simulink model "homeMobileManipulator"  (R2026a)
settings: Solver=ode4  StartTime=0  StopTime=Inf  FixedStep=cfg.rates.plant  MaxStep=cfg.rates.plant  AbsTol=1e-8
PostLoadFcn:
  | hmmSetup;
InitFcn:
  | hmmInitializeRun(bdroot);
values from neighbouring files (symbols this model uses):
  armJointLimits = zeros(numel(idx.arm), 2)    [hmmSetup.m]
  cfg = app.RunCfg    [HomeMobileManipulatorApp.m]    (also in HomeMobileManipulatorExample.m = params.cfg; hmmSetup.m = hmmConfig(); setupParams.m = data.cfg)
undefined symbols (not defined in the file or in its folder): actionQueueInit, actorNameTable, Angle, apertureMap, armPlanInit, Axis, basePlanInit, Custom, Extent, gray, gripperCoupling, invalidRayHits, movableRegistry, objectTargetInit, perceptionStatusInit, placeTargetInit, Position, robotStateInit, Sim3dSensor
libraries: robotmaniplib x20, robotcorelib x18, simulink x9, sim3dcameralib x6, sim3dgroundtruthsensorlib x4, dspmtrx3 x3, slpidlib x3, sim3dlib x3, hdlsllib x2, robotsim3dlib x1
(part 3 of 6)

== system homeMobileManipulator/MobileManipulator/Plant/RobotActor ==
  note: Scene frame -> render frame. The Simulation 3D Robot block negates y on EVERY LINK of
      | the tree it is given, while every Simulation 3D Actor and Camera here takes its
      | Translation as given - so the conversion is one frame change too many. RobotTree is
      | therefore handed renderRobot, a y-mirrored COPY of the tree (hmmMirrorTree), and driven
      | with the TRUE configuration: FK of the mirrored tree is M*FK(q)*M for every q, so the
      | block's own negation cancels exactly. This replaces a Gain that pre-negated the base y
      | and yaw only, which fixed 3 of 15 degrees of freedom and left the arm rendering as its
      | own mirror image. RENDER PATH ONLY - renderRobot's joint angles do not mean what they
      | say and its frames are left-handed; control, planning, perception and every FK
      | measurement use data.robot.
  GripperJointVector : Inport
  ArmJointPos : Inport  Port=2
  BasePose : Inport  Port=3
  TargetActorId : Inport  Port=4
  ActivateGrasp : Inport  Port=5
  TargetActorName : Inport  Port=6
  ActorRotationCol : Reshape  OutputDimensionality=Customize  OutputDimensions=[3 1]
  ActorTranslationCol : Reshape  OutputDimensionality=Customize  OutputDimensions=[3 1]
  AttachedActorSelect : Switch  Criteria=u2 ~= 0
  ConfigMux : Mux  Inputs=3
  ConfigRow : Reshape  OutputDimensionality=Customize  OutputDimensions=[1 15]
  NoActor : Constant  Value=cfg.actor.noneId  OutDataTypeStr=uint8
  ReleaseSettle : MATLAB Function  TreatAsAtomicUnit=on  SystemSampleTime=cfg.rates.scene
  RobotTree : robotsim3dlib/Simulation 3D Robot  actorInputType=RigidBodyTree Object  RigidBodyTree=renderRobot  ActorName=SimulinkVehicle1  existActorChekBox=off  initialTrans=[0 0 0]  initialRot=[0 0 0]  initialConfig=[cfg.base.initialPose(:)', cfg.arm.stowConfig, zeros(1,6)]  EndEffector=tcp_frame  eeOffsetInpChekBox=off  eeTargetTrans=carryTranslation  eeTargetRot=[0 0 0]  enableRegionGraspChekBox=off  regionGraspInpChekBox=off  eeTargTransDiff=[0.2 0.2 0.2]  eeTargRotDiff=[0 0 0]  enableVisualVisualization=on  enableCollisionVisualization=off  collisionGeomColor=[0 1 0]  collisionGeomTransp=0.1  inpConfEnbVal=on  inpGraspEnbVal=on  inpTransEnbVal=off  outConfEnbVal=off  outGraspEnbVal=on  outTransEnbVal=on  SampleTime=cfg.rates.scene  ActorType=SimulinkVehicle  ID=1  aMode=6  ActorTag=SimulinkVehicle1  Mesh=RigidBodyTree
      link override MATLAB System: RobotActorName=ActorName  EndEffectorName=EndEffector
  SettleDzOpen : Terminator
  RobotConfig : Outport
  ActorTranslation : Outport  Port=2
  ActorRotation : Outport  Port=3
  IsGrasped : Outport  Port=4
  AttachedActorId : Outport  Port=5
  wires:
  ActorRotationCol/1 -> ActorRotation/1  "ActorRotation"
  ActorTranslationCol/1 -> ActorTranslation/1  "ActorTranslation"
  AttachedActorSelect/1 -> AttachedActorId/1  "AttachedActorId"
  RobotTree/3 -> ActorRotationCol/1  "ActorRotationRow"
  RobotTree/2 -> ActorTranslationCol/1  "ActorTranslationRow"
  RobotTree/1 -> ReleaseSettle/1(IsGrasped), AttachedActorSelect/2, IsGrasped/1  "IsGrasped"
  TargetActorId/1 -> AttachedActorSelect/1, ReleaseSettle/2(TargetActorId)
  NoActor/1 -> AttachedActorSelect/3
  TargetActorName/1 -> RobotTree/2  "TargetActorName"
  ConfigRow/1 -> RobotTree/1, ReleaseSettle/3(RobotConfig), RobotConfig/1  "RobotConfig"
  ConfigMux/1 -> ConfigRow/1
  ActivateGrasp/1 -> RobotTree/3
  GripperJointVector/1 -> ConfigMux/3
  ArmJointPos/1 -> ConfigMux/2
  BasePose/1 -> ConfigMux/1
  ReleaseSettle/1(SettleDz) -> SettleDzOpen/1

== system homeMobileManipulator/MobileManipulator/Plant/StateReport ==
  BasePose : Inport
  BaseTwist : Inport  Port=2
  WheelSpeeds : Inport  Port=3
  ArmJointPos : Inport  Port=4
  ArmJointVel : Inport  Port=5
  GripperAperture : Inport  Port=6
  GripperDriverAngle : Inport  Port=7
  ToolTranslation : Inport  Port=8
  ToolRotation : Inport  Port=9
  ActorTranslation : Inport  Port=10
  ActorRotation : Inport  Port=11
  AttachedActorId : Inport  Port=12
  IsGrasped : Inport  Port=13
  ReportTime : DigitalClock  SampleTime=cfg.rates.plant
  RobotStateBus : BusCreator  Inputs=15  OutDataTypeStr=Bus: RobotState
      settings: InheritFromInputs=off
  StateValid : Constant  OutDataTypeStr=boolean
  RobotState : Outport
  wires:
  StateValid/1 -> RobotStateBus/15
  ReportTime/1 -> RobotStateBus/14
  IsGrasped/1 -> RobotStateBus/13
  AttachedActorId/1 -> RobotStateBus/12
  ActorRotation/1 -> RobotStateBus/11
  ActorTranslation/1 -> RobotStateBus/10
  ToolRotation/1 -> RobotStateBus/9
  ToolTranslation/1 -> RobotStateBus/8
  ArmJointVel/1 -> RobotStateBus/5
  ArmJointPos/1 -> RobotStateBus/4
  WheelSpeeds/1 -> RobotStateBus/3
  GripperDriverAngle/1 -> RobotStateBus/7
  BaseTwist/1 -> RobotStateBus/2
  GripperAperture/1 -> RobotStateBus/6
  BasePose/1 -> RobotStateBus/1
  RobotStateBus/1 -> RobotState/1

== system homeMobileManipulator/MobileManipulator/Plant/ToolKinematics ==
  RobotConfig : Inport
  GraspFramePose : robotmaniplib/Get Transform  RigidBodyTree=robot  SourceBody=grasp_frame  TargetBody=map  SimulateUsing=Code generation
  GraspRotationUnused : Terminator
  GraspToEuler : robotcorelib/Coordinate Transformation Conversion  InputRepresentation=Homogeneous Transformation  InputEulerSequence=ZYX  ShowTrVecInputPort=on  OutputRepresentation=Euler Angles  OutputEulerSequence=XYZ  ShowTrVecOutputPort=on  SimulateUsing=Code generation
  TcpPose : robotmaniplib/Get Transform  RigidBodyTree=robot  SourceBody=tcp_frame  TargetBody=map  SimulateUsing=Code generation
  TcpToEuler : robotcorelib/Coordinate Transformation Conversion  InputRepresentation=Homogeneous Transformation  InputEulerSequence=ZYX  ShowTrVecInputPort=on  OutputRepresentation=Euler Angles  OutputEulerSequence=XYZ  ShowTrVecOutputPort=on  SimulateUsing=Code generation
  ToolTranslation : Outport
  ToolRotation : Outport  Port=2
  GraspFramePos : Outport  Port=3
  wires:
  GraspToEuler/1 -> GraspRotationUnused/1
  TcpToEuler/1 -> ToolRotation/1  "ToolRotation"
  GraspFramePose/1 -> GraspToEuler/1  "GraspTransform"
  TcpPose/1 -> TcpToEuler/1  "TcpTransform"
  TcpToEuler/2 -> ToolTranslation/1  "ToolTranslation"
  RobotConfig/1 -> TcpPose/1, GraspFramePose/1
  GraspToEuler/2 -> GraspFramePos/1  "GraspFramePos"

== system homeMobileManipulator/MobileManipulator/SafetyMonitor/BaseLimitChecks ==
  BaseTwist : Inport
  AbsAccel : Abs
  AbsTwist : Abs
  AccelExceeded : RelationalOperator  Operator=>
  AccelLimits : Constant  Value=[cfg.base.axMax; cfg.base.ayMax; cfg.base.alphaMax]
  AnyBaseAccel : Logic  Operator=OR  Inputs=1  IconShape=distinctive
  AnyBaseVel : Logic  Operator=OR  Inputs=1  IconShape=distinctive
  BaseAccelEstimate : simulink/Discrete/Discrete Derivative  gainval=1  ICPrevScaledInput=0  OutMin=[]  OutMax=[]  OutDataType=fixdt(1, 16)  OutScaling=2^-10  DoSatur=off
  TwistLimits : Constant  Value=[cfg.base.vxMax; cfg.base.vyMax; cfg.base.omegaMax]
  VelExceeded : RelationalOperator  Operator=>
  BaseVel : Outport
  BaseAccel : Outport  Port=2
  wires:
  AnyBaseAccel/1 -> BaseAccel/1
  AnyBaseVel/1 -> BaseVel/1
  AccelLimits/1 -> AccelExceeded/2
  VelExceeded/1 -> AnyBaseVel/1  "VelExceeded"
  AbsAccel/1 -> AccelExceeded/1  "AbsAccel"
  TwistLimits/1 -> VelExceeded/2
  AbsTwist/1 -> VelExceeded/1  "AbsTwist"
  BaseAccelEstimate/1 -> AbsAccel/1
  BaseTwist/1 -> BaseAccelEstimate/1, AbsTwist/1
  AccelExceeded/1 -> AnyBaseAccel/1  "AccelExceeded"

== system homeMobileManipulator/MobileManipulator/SafetyMonitor/CausePriority ==
  Flags : Inport
  CauseCodes : Constant  Value=[cfg.sup.cause.JOINT_LIMIT; cfg.sup.cause.JOINT_VEL; cfg.sup.cause.JOINT_ACCEL; cfg.sup.cause.WORKSPACE; cfg.sup.cause.BASE_VEL; cfg.sup.cause.BASE_ACCEL; cfg.sup.cause.STALE_STATE; cfg.sup.cause.STALE_PLAN; cfg.sup.cause.STALE_PROVIDER]
  CauseSelect : Switch  Criteria=u2 ~= 0
  CodePerFlag : Switch  Criteria=u2 ~= 0
  FaultRaised : simulink/Logic and Bit Operations/Compare To Constant  relop=<=  const=cfg.sup.cause.nCauses  OutDataTypeStr=boolean
  LowestCode : MinMax
  NoCause : Constant  Value=uint8(cfg.sup.cause.NONE)
  NotRaised : Constant  Value=uint8(255 * ones(cfg.sup.cause.nCauses, 1))
  Cause : Outport
  AnyFault : Outport  Port=2
  wires:
  FaultRaised/1 -> AnyFault/1, CauseSelect/2
  LowestCode/1 -> FaultRaised/1, CauseSelect/1  "LowestCode"
  CodePerFlag/1 -> LowestCode/1
  NoCause/1 -> CauseSelect/3
  NotRaised/1 -> CodePerFlag/3
  CauseSelect/1 -> Cause/1
  Flags/1 -> CodePerFlag/2
  CauseCodes/1 -> CodePerFlag/1

== system homeMobileManipulator/MobileManipulator/SafetyMonitor/EStopLatch ==
  AnyFault : Inport
  Cause : Inport  Port=2
  CauseHold : UnitDelay  InitialCondition=uint8(cfg.sup.cause.NONE)  SampleTime=-1
  CauseSelect : Switch  Criteria=u2 ~= 0
  EStopPrev : UnitDelay  InitialCondition=false  SampleTime=-1
  Latch : Logic  Operator=OR  IconShape=distinctive
  EStop : Outport
  LatchedCause : Outport  Port=2
  wires:
  CauseHold/1 -> CauseSelect/1
  CauseSelect/1 -> CauseHold/1, LatchedCause/1
  Cause/1 -> CauseSelect/3
  Latch/1 -> EStop/1, EStopPrev/1
  AnyFault/1 -> Latch/1
  EStopPrev/1 -> Latch/2, CauseSelect/2

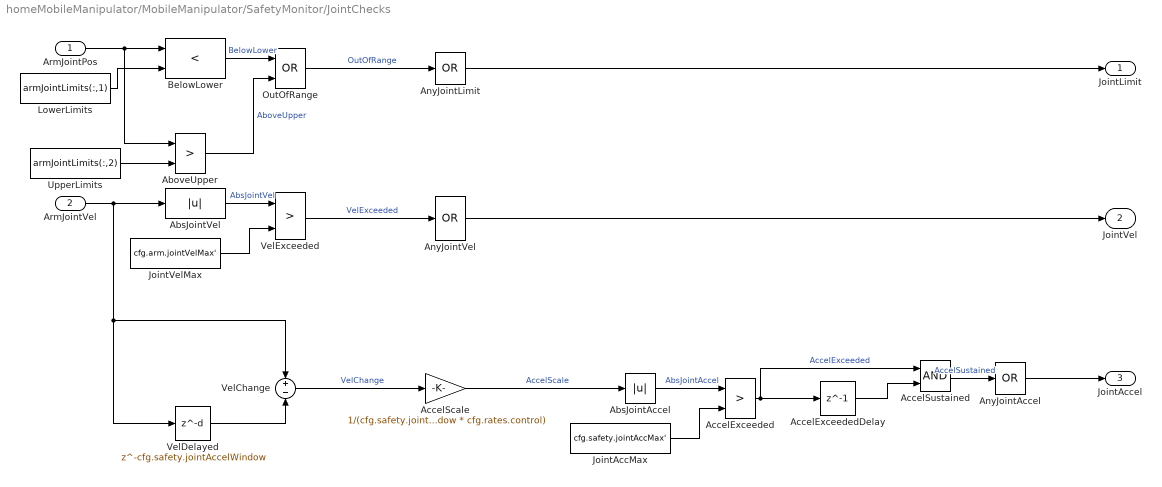
== system homeMobileManipulator/MobileManipulator/SafetyMonitor/JointChecks ==
  ArmJointPos : Inport
  ArmJointVel : Inport  Port=2
  AboveUpper : RelationalOperator  Operator=>
  AbsJointAccel : Abs
  AbsJointVel : Abs
  AccelExceeded : RelationalOperator  Operator=>
  AccelExceededDelay : Delay  DelayLength=1  InitialCondition=0
  AccelScale : Gain  Gain=1/(cfg.safety.jointAccelWindow * cfg.rates.control)
  AccelSustained : Logic  AllPortsSameDT=off  OutDataTypeStr=boolean
  AnyJointAccel : Logic  Operator=OR  Inputs=1  IconShape=distinctive
  AnyJointLimit : Logic  Operator=OR  Inputs=1  IconShape=distinctive
  AnyJointVel : Logic  Operator=OR  Inputs=1  IconShape=distinctive
  BelowLower : RelationalOperator  Operator=<
  JointAccMax : Constant  Value=cfg.safety.jointAccMax'
  JointVelMax : Constant  Value=cfg.arm.jointVelMax'
  LowerLimits : Constant  Value=armJointLimits(:,1)
  OutOfRange : Logic  Operator=OR  IconShape=distinctive
  UpperLimits : Constant  Value=armJointLimits(:,2)
  VelChange : Sum  Inputs=+-
  VelDelayed : Delay  DelayLength=cfg.safety.jointAccelWindow
  VelExceeded : RelationalOperator  Operator=>
  JointLimit : Outport
  JointVel : Outport  Port=2
  JointAccel : Outport  Port=3
  wires:
  AnyJointAccel/1 -> JointAccel/1
  AccelSustained/1 -> AnyJointAccel/1  "AccelSustained"
  AccelExceededDelay/1 -> AccelSustained/2
  AccelExceeded/1 -> AccelExceededDelay/1, AccelSustained/1  "AccelExceeded"
  JointAccMax/1 -> AccelExceeded/2
  AbsJointAccel/1 -> AccelExceeded/1  "AbsJointAccel"
  AccelScale/1 -> AbsJointAccel/1  "AccelScale"
  AnyJointVel/1 -> JointVel/1
  AnyJointLimit/1 -> JointLimit/1
  VelChange/1 -> AccelScale/1  "VelChange"
  VelExceeded/1 -> AnyJointVel/1  "VelExceeded"
  OutOfRange/1 -> AnyJointLimit/1  "OutOfRange"
  VelDelayed/1 -> VelChange/2
  AboveUpper/1 -> OutOfRange/2  "AboveUpper"
  ArmJointVel/1 -> VelDelayed/1, VelChange/1, AbsJointVel/1
  UpperLimits/1 -> AboveUpper/2
  AbsJointVel/1 -> VelExceeded/1  "AbsJointVel"
  JointVelMax/1 -> VelExceeded/2
  BelowLower/1 -> OutOfRange/1  "BelowLower"
  LowerLimits/1 -> BelowLower/2
  ArmJointPos/1 -> BelowLower/1, AboveUpper/1

== system homeMobileManipulator/MobileManipulator/SafetyMonitor/StalenessCheck ==
  RobotState : Inport
  BaseStatus : Inport  Port=2
  ArmStatus : Inport  Port=3
  PerceptionStatus : Inport  Port=4
  Now : Inport  Port=5
  ArmSelect : BusSelector  OutputSignals=Timestamp,Valid
  ArmStale : Subsystem  Description=|
      | Stale = (Now - Timestamp > Timeout) AND Fresh.
      | 
      | The Fresh gate is what stops this test from being a false alarm generator. Every timestamp on every bus starts at the ground value 0, so an ungated age test fires on EVERY producer at t = Timeout, before the producer has run once, and a latched e-stop would kill the run before the task starts. Fresh says "this producer is supposed to be reporting right now": Valid for the state and status buses, State == pending for the grounding provider, whose timestamp legitimately freezes once the one request it makes has completed.
  BaseSelect : BusSelector  OutputSignals=Timestamp,Valid
  BaseStale : Subsystem  Description=|
      | Stale = (Now - Timestamp > Timeout) AND Fresh.
      | 
      | The Fresh gate is what stops this test from being a false alarm generator. Every timestamp on every bus starts at the ground value 0, so an ungated age test fires on EVERY producer at t = Timeout, before the producer has run once, and a latched e-stop would kill the run before the task starts. Fresh says "this producer is supposed to be reporting right now": Valid for the state and status buses, State == pending for the grounding provider, whose timestamp legitimately freezes once the one request it makes has completed.
  PlanStale : Logic  Operator=OR  IconShape=distinctive
  ProviderSelect : BusSelector  OutputSignals=State,Timestamp
  ProviderStale : Subsystem  Description=|
      | Stale = (Now - Timestamp > Timeout) AND Fresh.
      | 
      | The Fresh gate is what stops this test from being a false alarm generator. Every timestamp on every bus starts at the ground value 0, so an ungated age test fires on EVERY producer at t = Timeout, before the producer has run once, and a latched e-stop would kill the run before the task starts. Fresh says "this producer is supposed to be reporting right now": Valid for the state and status buses, State == pending for the grounding provider, whose timestamp legitimately freezes once the one request it makes has completed.
  ProviderTimeout : Constant  Value=cfg.provider.timeout
  RequestPending : simulink/Logic and Bit Operations/Compare To Constant  relop===  const=uint8(1)  OutDataTypeStr=boolean
  StaleTimeout : Constant  Value=cfg.safety.staleTimeout
  StateSelect : BusSelector  OutputSignals=Timestamp,Valid
  StateStale : Subsystem  Description=|
      | Stale = (Now - Timestamp > Timeout) AND Fresh.
      | 
      | The Fresh gate is what stops this test from being a false alarm generator. Every timestamp on every bus starts at the ground value 0, so an ungated age test fires on EVERY producer at t = Timeout, before the producer has run once, and a latched e-stop would kill the run before the task starts. Fresh says "this producer is supposed to be reporting right now": Valid for the state and status buses, State == pending for the grounding provider, whose timestamp legitimately freezes once the one request it makes has completed.
  StaleState : Outport
  StalePlan : Outport  Port=2
  StaleProvider : Outport  Port=3
  wires:
  ProviderStale/1(Stale) -> StaleProvider/1
  BaseStale/1(Stale) -> PlanStale/1
  PlanStale/1 -> StalePlan/1
  RequestPending/1 -> ProviderStale/4(Fresh)
  ArmStale/1(Stale) -> PlanStale/2
  ProviderTimeout/1 -> ProviderStale/3(Timeout)
  StateSelect/2 -> StateStale/4(Fresh)  "<Valid>"
  Now/1 -> StateStale/1(Now), ArmStale/1(Now), BaseStale/1(Now), ProviderStale/1(Now)
  ArmSelect/2 -> ArmStale/4(Fresh)  "<Valid>"
  ArmSelect/1 -> ArmStale/2(Timestamp)  "<Timestamp>"
  BaseSelect/2 -> BaseStale/4(Fresh)  "<Valid>"
  StaleTimeout/1 -> BaseStale/3(Timeout), ArmStale/3(Timeout), StateStale/3(Timeout)
  ProviderSelect/2 -> ProviderStale/2(Timestamp)  "<Timestamp>"
  ProviderSelect/1 -> RequestPending/1  "<State>"
  RobotState/1 -> StateSelect/1
  StateSelect/1 -> StateStale/2(Timestamp)  "<Timestamp>"
  ArmStatus/1 -> ArmSelect/1
  BaseStatus/1 -> BaseSelect/1
  BaseSelect/1 -> BaseStale/2(Timestamp)  "<Timestamp>"
  PerceptionStatus/1 -> ProviderSelect/1
  StateStale/1(Stale) -> StaleState/1

== system homeMobileManipulator/MobileManipulator/SafetyMonitor/WorkspaceCheck ==
  ArmJointPos : Inport
  ToolTranslation : Inport  Port=2
  AboveBounds : RelationalOperator  Operator=>
  AnyOutOfBounds : Logic  Operator=OR  Inputs=1  IconShape=distinctive
  BelowBounds : RelationalOperator  Operator=<
  BoundsMax : Constant  Value=cfg.percep.sceneBounds(:,2)
  BoundsMin : Constant  Value=cfg.percep.sceneBounds(:,1)
  OutOfBounds : Logic  Operator=OR  IconShape=distinctive
  ReachExceeded : simulink/Logic and Bit Operations/Compare To Constant  relop=>  const=cfg.safety.toolReachMax  OutDataTypeStr=boolean
  ReachNorm : Sqrt  Description=|
      | Euclidean distance from arm_mount to the tool, compared against cfg.arm.reach by ReachExceeded.
      | 
      | Operator MUST be sqrt. It was rSqrt - the RECIPROCAL square root - which inverts the comparison and reads 2.258 for the stow pose's 0.443 m, so the reach check tripped on every step of every run and latched the e-stop. The two spellings are indistinguishable on the canvas and the block accepts either without complaint.
  ReachSq : DotProduct
  ToolPoseInArmFrame : Subsystem
  WorkspaceViolation : Logic  Operator=OR  IconShape=distinctive
  Workspace : Outport
  wires:
  WorkspaceViolation/1 -> Workspace/1
  AnyOutOfBounds/1 -> WorkspaceViolation/2  "AnyOutOfBounds"
  OutOfBounds/1 -> AnyOutOfBounds/1  "OutOfBounds"
  ReachNorm/1 -> ReachExceeded/1  "ReachNorm"
  ReachExceeded/1 -> WorkspaceViolation/1
  ReachSq/1 -> ReachNorm/1  "ReachSq"
  AboveBounds/1 -> OutOfBounds/2  "AboveBounds"
  BelowBounds/1 -> OutOfBounds/1  "BelowBounds"
  BoundsMax/1 -> AboveBounds/2
  ToolPoseInArmFrame/1(ToolTranslation) -> ReachSq/1, ReachSq/2
  ToolTranslation/1 -> BelowBounds/1, AboveBounds/1
  ArmJointPos/1 -> ToolPoseInArmFrame/1(ArmConfig)
  BoundsMin/1 -> BelowBounds/2

== system homeMobileManipulator/Perception/SceneGrounding/Grounding ==
  CameraFrames : Inport  OutDataTypeStr=Bus: CameraFrame  PortDimensions=5
  TaskRequest : Inport  Port=2  OutDataTypeStr=Bus: TaskRequest
  SimTime : Inport  Port=3
  ActiveIndex : Inport  Port=4  OutDataTypeStr=uint8
  GroundingService : MATLAB Function  Description=SIMULINK-FIRST JUSTIFICATION: no dedicated block exists. Searched robotlib, robotmaniplib, navlib and visionlib with find_system(lib,'SearchDepth',2,'Type','Block'); none provides an HTTP request, base64 PNG encoding or JSON decoding. No native Simulink equivalent exists either - webwrite, jsondecode and matlab.net.base64encode have no block form at all, so the native block count is not large, it is undefined. Rung 4 of the ladder is the only rung.  TreatAsAtomicUnit=on
  NextRequestId : Bias  Bias=1
  PrevQueue : UnitDelay  InitialCondition=actionQueueInit  SampleTime=-1
  QueueFailure : BusSelector  OutputSignals=FailureCode
  RequestId : DataTypeConversion  OutDataTypeStr=uint32  SaturateOnIntegerOverflow=off  RndMeth=Floor
  RequestIdState : UnitDelay  SampleTime=-1
  Status : BusCreator  Inputs=10  OutDataTypeStr=Bus: PerceptionStatus  NonVirtualBus=on
      settings: InheritFromInputs=off
  StatusValid : Constant  Value=true  OutDataTypeStr=boolean
  TaskId : BusSelector  OutputSignals=TaskId
  ActionQueue : Outport  OutDataTypeStr=Bus: ActionQueue
  PerceptionStatus : Outport  Port=2  OutDataTypeStr=Bus: PerceptionStatus
  wires:
  Status/1 -> PerceptionStatus/1
  QueueFailure/1 -> Status/8  "<FailureCode>"
  GroundingService/5(Latency) -> Status/6
  GroundingService/6(NumActions) -> Status/7
  GroundingService/3(State) -> Status/4
  GroundingService/4(HttpStatus) -> Status/5
  GroundingService/1(ActionQueue) -> PrevQueue/1, QueueFailure/1, ActionQueue/1
  GroundingService/2(Route) -> Status/3
  TaskId/1 -> Status/2  "<TaskId>"
  SimTime/1 -> GroundingService/4(simTime), Status/9
  ActiveIndex/1 -> GroundingService/6(activeIndex)
  CameraFrames/1 -> GroundingService/1(frames)
  RequestId/1 -> RequestIdState/1, GroundingService/3(requestId), Status/1  "RequestId"
  StatusValid/1 -> Status/10  "Valid"
  RequestIdState/1 -> NextRequestId/1
  PrevQueue/1 -> GroundingService/5(queueTemplate)
  TaskRequest/1 -> GroundingService/2(task), TaskId/1
  NextRequestId/1 -> RequestId/1  "NextRequestId"

== system homeMobileManipulator/Perception/SceneGrounding/Reconstruction ==
  CameraFrames : Inport  OutDataTypeStr=Bus: CameraFrame  PortDimensions=5
  ActionQueue : Inport  Port=2  OutDataTypeStr=Bus: ActionQueue
  MovableRegistry : Inport  Port=3  OutDataTypeStr=Bus: MovableRegistry
  SimTime : Inport  Port=4
  ObjectTemplate : Constant  Value=objectTargetInit  OutDataTypeStr=Bus: ObjectTarget
  PlaceTemplate : Constant  Value=placeTargetInit  OutDataTypeStr=Bus: PlaceTarget
  TargetReconstruction : MATLAB Function  Description=SIMULINK-FIRST JUSTIFICATION: no dedicated block exists. Searched visionlib, robotlib, robotmaniplib and navlib with find_system(lib,'SearchDepth',2,'Type','Block'); Computer Vision Toolbox ships no plane-fit block and no pointCloud block, and there is no block form of pcfitplane. A native Simulink equivalent would need the RANSAC consensus loop, the per-camera ray-window search, the actor association test and the 3x3 principal-axis decomposition - estimated well over 80 blocks, and the RANSAC iteration count is data dependent, which a fixed block diagram cannot express at all.  TreatAsAtomicUnit=on
  ObjectTarget : Outport  OutDataTypeStr=Bus: ObjectTarget
  PlaceTarget : Outport  Port=2  OutDataTypeStr=Bus: PlaceTarget
  wires:
  TargetReconstruction/2(plc) -> PlaceTarget/1
  PlaceTemplate/1 -> TargetReconstruction/6(plcTemplate)
  ObjectTemplate/1 -> TargetReconstruction/5(objTemplate)
  SimTime/1 -> TargetReconstruction/4(simTime)
  MovableRegistry/1 -> TargetReconstruction/3(registry)
  ActionQueue/1 -> TargetReconstruction/2(queue)
  TargetReconstruction/1(obj) -> ObjectTarget/1
  CameraFrames/1 -> TargetReconstruction/1(frames)

== system homeMobileManipulator/Perception/SceneGrounding/SceneMapping ==
  CameraFrames : Inport  OutDataTypeStr=Bus: CameraFrame  PortDimensions=5
  RobotState : Inport  Port=2  OutDataTypeStr=Bus: RobotState
  BasePoseSelect : BusSelector  OutputSignals=BasePose
  GridIn : DataStoreRead  DataStoreName=NavMapGrid  IndexOptions=Index vector (dialog)  Indices=1  OutputSizes=1
  GridOut : DataStoreWrite  DataStoreName=NavMapGrid  IndexOptions=Index vector (dialog)  Indices=1  OutputSizes=1
  MapUpdate : MATLAB Function  Description=SIMULINK-FIRST JUSTIFICATION: no dedicated block exists. Searched navlib with find_system('navlib','SearchDepth',2,'Type','Block'); Navigation Toolbox provides no occupancyMap block and no updateOccupancy block - the map is a handle object with no block form. A native equivalent would have to reimplement log-odds accumulation, world-to-grid indexing and the per-call duplicate collapse over a 240x240 grid; that is not a 15-block diagram, and a second implementation of the map arithmetic is exactly the drift this project forbids.  TreatAsAtomicUnit=on
  wires:
  GridIn/1 -> MapUpdate/3(priorGrid)
  MapUpdate/1(grid) -> GridOut/1
  BasePoseSelect/1 -> MapUpdate/2(basePose)  "<BasePose>"
  CameraFrames/1 -> MapUpdate/1(frames)
  RobotState/1 -> BasePoseSelect/1

== system homeMobileManipulator/MobileManipulator/Manipulator/ArmControl/ApproachReference ==
  TargetPose : Inport
  ArmJointPos : Inport  Port=2
  ApproachIK : robotmaniplib/Inverse Kinematics  Description=|  RigidBodyTree=armIkTree  EndEffector=tcp_frame  ShowInfo=off  SolverName=BFGS Gradient Projection  EnforceJointLimits=on  AllowRandomRestarts=off  MaxIterations=cfg.plan.ikMaxIterations  MaxTime=cfg.plan.ikMaxTime  GradientTolerance=1e-7  SolutionTolerance=1e-6  StepTolerance=1e-14  ConstraintTolerance=1e-6  ErrorChangeTolerance=1e-12  UseErrorDamping=on  DampingBias=0.0025  RandomStream=Global stream  Seed=cfg.plan.ikSeed  SimulateUsing=Code generation
      | IK on armIkTree to tcp_frame, the SAME tree and end effector ApproachTarget/GraspTransform uses, so the 4x4 it is handed and the 4x4 GetTransform produces are the same quantity in the same frame - armIkTree's base is arm_mount, which is GetTransform's TargetBody.
      | 
      | AllowRandomRestarts is OFF, and that is the whole point. A random restart is licence to return a DIFFERENT BRANCH than the seed, which is exactly the failure this block was added to remove. cfg.plan.ikWeights is reused rather than restated so the reference is screened on the same terms the grasp candidates were.
      | 
      | Config comes out 12x1 - 6 arm joints then 6 gripper joints, in armIkTree's non-fixed joint order - despite the tree's DataFormat being 'row'. ArmJointSelect takes the arm six.
  ArmJointSelect : Gain  Gain=[eye(cfg.arm.nJoints), zeros(cfg.arm.nJoints, cfg.gripper.nJoints)]  Multiplication=Matrix(K*u)
  FullGuess : Mux  Description=[measured arm configuration; gripper zeros] as the IK seed. The gripper joints are padded to zero because armIkTree carries all twelve and the approach does not move the fingers - GripperDriver owns those.  Inputs=2
  GripperZero : Constant  Value=zeros(cfg.gripper.nJoints, 1)
  IkWeights : Constant  Value=cfg.plan.ikWeights
  RefPos : Outport
  wires:
  GripperZero/1 -> FullGuess/2
  ArmJointPos/1 -> FullGuess/1
  TargetPose/1 -> ApproachIK/1
  IkWeights/1 -> ApproachIK/2
  FullGuess/1 -> ApproachIK/3  "IkGuess"
  ApproachIK/1 -> ArmJointSelect/1  "IkConfig"
  ArmJointSelect/1 -> RefPos/1

== system homeMobileManipulator/MobileManipulator/Manipulator/ArmControl/ApproachTarget ==
  GraspConfig : Inport
  ApproachOffset : Inport  Port=2
  ConfigRow : Math  Operator=transpose
  FullConfig : Mux  Inputs=2
  GraspTransform : robotmaniplib/Get Transform  RigidBodyTree=armIkTree  SourceBody=tcp_frame  TargetBody=arm_mount  SimulateUsing=Code generation
  GripperZero : Constant  Value=zeros(cfg.gripper.nJoints, 1)
  OffsetNegative : Gain  Gain=[0;0;-1]
  OffsetTransform : robotcorelib/Coordinate Transformation Conversion  InputRepresentation=Translation Vector  InputEulerSequence=ZYX  ShowTrVecInputPort=off  OutputRepresentation=Homogeneous Transformation  OutputEulerSequence=ZYX  ShowTrVecOutputPort=off  SimulateUsing=Code generation
  TargetPoseProduct : Product  Multiplication=Matrix(*)
  TranslationSelect : robotcorelib/Coordinate Transformation Conversion  InputRepresentation=Homogeneous Transformation  InputEulerSequence=ZYX  ShowTrVecInputPort=off  OutputRepresentation=Translation Vector  OutputEulerSequence=ZYX  ShowTrVecOutputPort=off  SimulateUsing=Code generation
  TargetPose : Outport
  TargetTranslation : Outport  Port=2
  wires:
  TranslationSelect/1 -> TargetTranslation/1
  ConfigRow/1 -> GraspTransform/1  "ConfigRow"
  OffsetNegative/1 -> OffsetTransform/1  "OffsetNegative"
  FullConfig/1 -> ConfigRow/1  "FullConfig"
  GripperZero/1 -> FullConfig/2
  ApproachOffset/1 -> OffsetNegative/1
  GraspConfig/1 -> FullConfig/1
  TargetPoseProduct/1 -> TargetPose/1, TranslationSelect/1  "TargetPoseProduct"
  OffsetTransform/1 -> TargetPoseProduct/2
  GraspTransform/1 -> TargetPoseProduct/1

== system homeMobileManipulator/MobileManipulator/Manipulator/ArmControl/JointSpaceTrack ==
  RefPosNow : Inport
  RefVelNow : Inport  Port=2
  JointAccelOpen : Terminator
  JointCmdColumn : Reshape  Description=|  OutputDimensionality=Column vector (2-D)
      | Makes the joint command an explicit [6 1] COLUMN.
      | 
      | This was a Math Function transpose, which is the obvious block and the wrong one:
      | the Joint Space Motion Model emits an UNORIENTED 1-D signal, and transposing a 1-D
      | signal yields a ROW, so this branch of the mode switch disagreed in orientation with
      | the task-space branch that arrives as [6 1]. Reshape states the orientation instead
      | of flipping whatever orientation happens to arrive.
  JointCmdLead : Sum
  JointSpaceMotionModel : robotmaniplib/Joint Space Motion Model  RigidBodyTree=armDynTree  MotionType=Independent Joint Motion  ProportionalGain=100  DerivativeGain=10  ErrorDynamicsSpecification=Damping Ratio / Natural Frequency  DampingRatio=cfg.track.armDampingRatio  NaturalFrequency=cfg.track.armNaturalFreq  SettlingTime=0.472  Overshoot=0  ShowExternalForcePort=off  InitConfig=cfg.arm.stowConfig  InitJointVel=zeros(1, cfg.arm.nJoints)  SimulateUsing=Code generation
  JointVelOpen : Terminator
  PlantLagLead : Gain  Gain=cfg.arm.jointTimeConst
  RefAccZero : Constant  Value=zeros(1, cfg.arm.nJoints)
  RefPosRow : Math  Operator=transpose
  RefVelRow : Math  Operator=transpose
  JointCmd : Outport
  wires:
  JointCmdLead/1 -> JointCmd/1  "JointCmdLead"
  JointCmdColumn/1 -> JointCmdLead/1
  PlantLagLead/1 -> JointCmdLead/2  "PlantLagLead"
  RefAccZero/1 -> JointSpaceMotionModel/3
  JointSpaceMotionModel/2 -> JointVelOpen/1
  RefVelRow/1 -> JointSpaceMotionModel/2  "RefVelRow"
  RefVelNow/1 -> RefVelRow/1, PlantLagLead/1
  JointSpaceMotionModel/3 -> JointAccelOpen/1
  RefPosNow/1 -> RefPosRow/1
  RefPosRow/1 -> JointSpaceMotionModel/1  "RefPosRow"
  JointSpaceMotionModel/1 -> JointCmdColumn/1

== system homeMobileManipulator/MobileManipulator/Manipulator/ArmControl/MeasuredToolPose ==
  ArmConfig : Inport
  ConfigRow : Math  Operator=transpose
  FullConfig : Mux  Inputs=2
  GripperZero : Constant  Value=zeros(cfg.gripper.nJoints, 1)
  ToolTransform : robotmaniplib/Get Transform  RigidBodyTree=armIkTree  SourceBody=tcp_frame  TargetBody=arm_mount  SimulateUsing=Code generation
  TranslationHomogeneous : Product  Multiplication=Matrix(*)
  TranslationPick : Constant  Value=[0;0;0;1]
  TranslationSelect : Gain  Gain=[eye(3), zeros(3,1)]  Multiplication=Matrix(K*u)
  ToolTranslation : Outport
  ToolPose : Outport  Description=The measured tool pose as a full 4x4, in the arm_mount frame. TaskSpaceTrack holds its internal model on this whenever task-space mode is not engaged, so the model tracks the real arm instead of integrating toward a target nobody asked for.  Port=2
  wires:
  TranslationSelect/1 -> ToolTranslation/1  "TranslationSelect"
  TranslationPick/1 -> TranslationHomogeneous/2
  ToolTransform/1 -> TranslationHomogeneous/1, ToolPose/1
  TranslationHomogeneous/1 -> TranslationSelect/1  "TranslationHomogeneous"
  ConfigRow/1 -> ToolTransform/1  "ConfigRow"
  FullConfig/1 -> ConfigRow/1  "FullConfig"
  ArmConfig/1 -> FullConfig/1
  GripperZero/1 -> FullConfig/2

== system homeMobileManipulator/MobileManipulator/Manipulator/ArmControl/ReferenceSample ==
  MoveTime : Inport
  Duration : Inport  Port=2
  RefTime : Inport  Port=3
  RefPos : Inport  Port=4
  RefVel : Inport  Port=5
  ClampTime : MinMax  Inputs=2
  RefAccelUnused : Terminator
  ReferenceTrajectory : robotcorelib/Polynomial Trajectory  Description=Robotics System Toolbox Polynomial Trajectory (cubic Hermite): the arm joint reference at MoveTime, through the planner's timed samples with its own velocities as boundary conditions. Replaces a hand-wired PreLookup + Direct Lookup Table linear blend (2026-10-08).  WaypointSource=External  Waypoints=[ 0, 2, 1, 5, 0; -1, 3, 1, 4, 4 ]  TimePoints=[ 0, 1, 2, 3, 4 ]  TimeInterval=[ 1, 4 ]  Method=Cubic Polynomial  ParameterSource=External  VelocityBoundaryCondition=zeros( 2, 5 )  AccelerationBoundaryCondition=zeros( 2, 5 )  SimulateUsing=Code generation
  RefPosNow : Outport
  RefVelNow : Outport  Port=2
  wires:
  ReferenceTrajectory/3 -> RefAccelUnused/1
  ReferenceTrajectory/2 -> RefVelNow/1
  ClampTime/1 -> ReferenceTrajectory/1  "ClampTime"
  Duration/1 -> ClampTime/2
  RefPos/1 -> ReferenceTrajectory/2
  RefTime/1 -> ReferenceTrajectory/3
  RefVel/1 -> ReferenceTrajectory/4
  MoveTime/1 -> ClampTime/1
  ReferenceTrajectory/1 -> RefPosNow/1

== system homeMobileManipulator/MobileManipulator/Manipulator/ArmControl/ReferenceSelect ==
  RefPosNow : Inport
  RefVelNow : Inport  Port=2
  StowSelect : Inport  Port=3
  TaskTrackEngaged : Inport  Port=4
  ApproachRefPos : Inport  Port=5
  HoldSelect : Inport  Port=6
  MeasuredPos : Inport  Port=7
  ApproachPositionSelect : Switch  Description=Three sources for one joint reference, in priority order: approach IK when TaskTrackEngaged, else stow when StowSelect, else the plan sample. The two flags are never both true - ArmSupervisor's Idle, Stowing and AwaitPlan set StowSelect with TaskSpaceMode false, and Retreating and ApproachConstrained set TaskSpaceMode with StowSelect false - so a chain of two switches is a total function and not a race.  Criteria=u2 ~= 0
  ApproachVelocity : Constant  Description=ZERO, DELIBERATELY, and here is the arithmetic. JointSpaceMotionModel is a critically damped tracker at cfg.track.armNaturalFreq = 12.5 rad/s, so with no velocity feedforward it lags a moving reference by about 2*zeta*v/wn. The approach target moves at approachRate = 3*cfg.sup.approachDepth/cfg.sup.timeout.approach = 0.03 m/s, giving a lag near 4.8 mm - well inside the 150 mm cfg.safety.trackErrMax guard, and it decays to nothing before it is ever tested, because the exit gate requires ApproachOffset to have REACHED depthTarget and the target is then static. Differentiating the IK output to get a real feedforward would buy 5 mm of transient at the cost of differentiating a solver's output.  Value=zeros(cfg.arm.nJoints, 1)
  ApproachVelocitySelect : Switch  Criteria=u2 ~= 0
  HoldPositionSelect : Switch  Criteria=u2 ~= 0  SaturateOnIntegerOverflow=off  InputSameDT=off
  HoldVelocitySelect : Switch  Criteria=u2 ~= 0  SaturateOnIntegerOverflow=off  InputSameDT=off
  PositionSelect : Switch  Criteria=u2 ~= 0  SaturateOnIntegerOverflow=off  InputSameDT=off
  StowConfig : Constant  Value=cfg.arm.stowConfig'
  StowVelocity : Constant  Value=zeros(cfg.arm.nJoints, 1)
  VelocitySelect : Switch  Criteria=u2 ~= 0  SaturateOnIntegerOverflow=off  InputSameDT=off
  RefPos : Outport
  RefVel : Outport  Port=2
  wires:
  ApproachVelocitySelect/1 -> RefVel/1
  ApproachPositionSelect/1 -> RefPos/1
  TaskTrackEngaged/1 -> ApproachVelocitySelect/2, ApproachPositionSelect/2
  HoldPositionSelect/1 -> ApproachPositionSelect/3
  VelocitySelect/1 -> HoldVelocitySelect/3
  StowVelocity/1 -> VelocitySelect/1, HoldVelocitySelect/1
  RefVelNow/1 -> VelocitySelect/3
  PositionSelect/1 -> HoldPositionSelect/3
  HoldSelect/1 -> HoldVelocitySelect/2, HoldPositionSelect/2
  StowConfig/1 -> PositionSelect/1
  ApproachRefPos/1 -> ApproachPositionSelect/1
  RefPosNow/1 -> PositionSelect/3
  StowSelect/1 -> VelocitySelect/2, PositionSelect/2
  HoldVelocitySelect/1 -> ApproachVelocitySelect/3
  MeasuredPos/1 -> HoldPositionSelect/1
  ApproachVelocity/1 -> ApproachVelocitySelect/1

== system homeMobileManipulator/MobileManipulator/Manipulator/ArmControl/ReferenceToolPose ==
  ArmConfig : Inport
  ConfigRow : Math  Operator=transpose
  FullConfig : Mux  Inputs=2
  GripperZero : Constant  Value=zeros(cfg.gripper.nJoints, 1)
  ToolTransform : robotmaniplib/Get Transform  RigidBodyTree=armIkTree  SourceBody=tcp_frame  TargetBody=arm_mount  SimulateUsing=Code generation
  TranslationHomogeneous : Product  Multiplication=Matrix(*)
  TranslationPick : Constant  Value=[0;0;0;1]
  TranslationSelect : Gain  Gain=[eye(3), zeros(3,1)]  Multiplication=Matrix(K*u)
  ToolTranslation : Outport
  wires:
  TranslationSelect/1 -> ToolTranslation/1  "TranslationSelect"
  TranslationPick/1 -> TranslationHomogeneous/2
  ToolTransform/1 -> TranslationHomogeneous/1
  ConfigRow/1 -> ToolTransform/1  "ConfigRow"
  FullConfig/1 -> ConfigRow/1  "FullConfig"
  GripperZero/1 -> FullConfig/2
  ArmConfig/1 -> FullConfig/1
  TranslationHomogeneous/1 -> TranslationSelect/1  "TranslationHomogeneous"

== system homeMobileManipulator/MobileManipulator/Manipulator/ArmControl/TrackingMetrics ==
  RefPosNow : Inport
  ArmJointPos : Inport  Port=2
  MeasuredToolTranslation : Inport  Port=3
  TargetTranslation : Inport  Port=4
  RefToolTranslation : Inport  Port=5
  TaskSpaceMode : Inport  Port=6
  JointErrorNorm : Sqrt
  JointErrorSquared : DotProduct  OutDataTypeStr=Inherit: Inherit via internal rule
  JointErrorVector : Sum  Inputs=+-
  SettledCheck : simulink/Logic and Bit Operations/Compare To Constant  relop=<=  const=cfg.arm.settleBand  OutDataTypeStr=boolean
  TargetSelect : Switch  Criteria=u2 ~= 0  SaturateOnIntegerOverflow=off  InputSameDT=off
  ToolErrorSquared : DotProduct  OutDataTypeStr=Inherit: Inherit via internal rule
  ToolErrorVector : Sum  Inputs=+-
  TrackingErrorNorm : Sqrt
  JointError : Outport
  TrackingError : Outport  Port=2
  Settled : Outport  Port=3
  wires:
  SettledCheck/1 -> Settled/1
  TrackingErrorNorm/1 -> TrackingError/1, SettledCheck/1
  ToolErrorSquared/1 -> TrackingErrorNorm/1  "ToolErrorSquared"
  ToolErrorVector/1 -> ToolErrorSquared/2, ToolErrorSquared/1  "ToolErrorVector"
  JointErrorSquared/1 -> JointErrorNorm/1  "JointErrorSquared"
  TargetSelect/1 -> ToolErrorVector/2
  MeasuredToolTranslation/1 -> ToolErrorVector/1
  JointErrorNorm/1 -> JointError/1
  JointErrorVector/1 -> JointErrorSquared/2, JointErrorSquared/1  "JointErrorVector"
  RefPosNow/1 -> JointErrorVector/2
  RefToolTranslation/1 -> TargetSelect/3
  TargetTranslation/1 -> TargetSelect/1
  TaskSpaceMode/1 -> TargetSelect/2
  ArmJointPos/1 -> JointErrorVector/1

== system homeMobileManipulator/MobileManipulator/Manipulator/MotionPlanning/CandidateIK ==
  GraspPoint : Inport
  TfArmFromMap : Inport  Port=2
  IkGuess : Inport  Port=3
  Candidate_1 : Subsystem
  Candidate_2 : Subsystem
  Candidate_3 : Subsystem
  ConfigCat : Concatenate  NumInputs=3  Mode=Multidimensional array  ConcatenateDimension=2
  ErrCat : Concatenate  NumInputs=3
  IkWeights : Constant  Value=cfg.plan.ikWeights
  ManipCat : Concatenate  NumInputs=3
  PoseCat : Concatenate  NumInputs=3  Mode=Multidimensional array  ConcatenateDimension=3
  GraspConfigs : Outport
  PoseErrors : Outport  Port=2
  Manipulability : Outport  Port=3
  GraspPoses : Outport  Port=4
  wires:
  PoseCat/1 -> GraspPoses/1
  ManipCat/1 -> Manipulability/1
  ErrCat/1 -> PoseErrors/1
  ConfigCat/1 -> GraspConfigs/1
  Candidate_3/4(GraspPose) -> PoseCat/3
  Candidate_3/3(Manipulability) -> ManipCat/3
  Candidate_3/2(PoseError) -> ErrCat/3
  Candidate_3/1(Config) -> ConfigCat/3
  Candidate_2/2(PoseError) -> ErrCat/2
  Candidate_1/4(GraspPose) -> PoseCat/1
  Candidate_1/2(PoseError) -> ErrCat/1
  Candidate_2/4(GraspPose) -> PoseCat/2
  IkWeights/1 -> Candidate_3/4(IkWeights), Candidate_2/4(IkWeights), Candidate_1/4(IkWeights)
  TfArmFromMap/1 -> Candidate_1/2(TfArmFromMap), Candidate_3/2(TfArmFromMap), Candidate_2/2(TfArmFromMap)
  Candidate_2/1(Config) -> ConfigCat/2
  Candidate_1/1(Config) -> ConfigCat/1
  GraspPoint/1 -> Candidate_1/1(GraspPoint), Candidate_2/1(GraspPoint), Candidate_3/1(GraspPoint)
  IkGuess/1 -> Candidate_1/3(IkGuess), Candidate_3/3(IkGuess), Candidate_2/3(IkGuess)
  Candidate_2/3(Manipulability) -> ManipCat/2
  Candidate_1/3(Manipulability) -> ManipCat/1

== system homeMobileManipulator/MobileManipulator/Manipulator/MotionPlanning/ConfigAssembly ==
  RobotState : Inport  OutDataTypeStr=Bus: RobotState
  ArmConfig : Concatenate
  FullConfig : Concatenate
  GripperZeros : Constant  Value=zeros(cfg.gripper.nJoints, 1)
  StateSelect : BusSelector  OutputSignals=BasePose,ArmJointPos
  RobotConfig : Outport
  IkGuess : Outport  Port=2
  wires:
  StateSelect/2 -> ArmConfig/1  "<ArmJointPos>"
  StateSelect/1 -> FullConfig/1  "<BasePose>"
  GripperZeros/1 -> ArmConfig/2
  RobotState/1 -> StateSelect/1
  ArmConfig/1 -> FullConfig/2, IkGuess/1
  FullConfig/1 -> RobotConfig/1

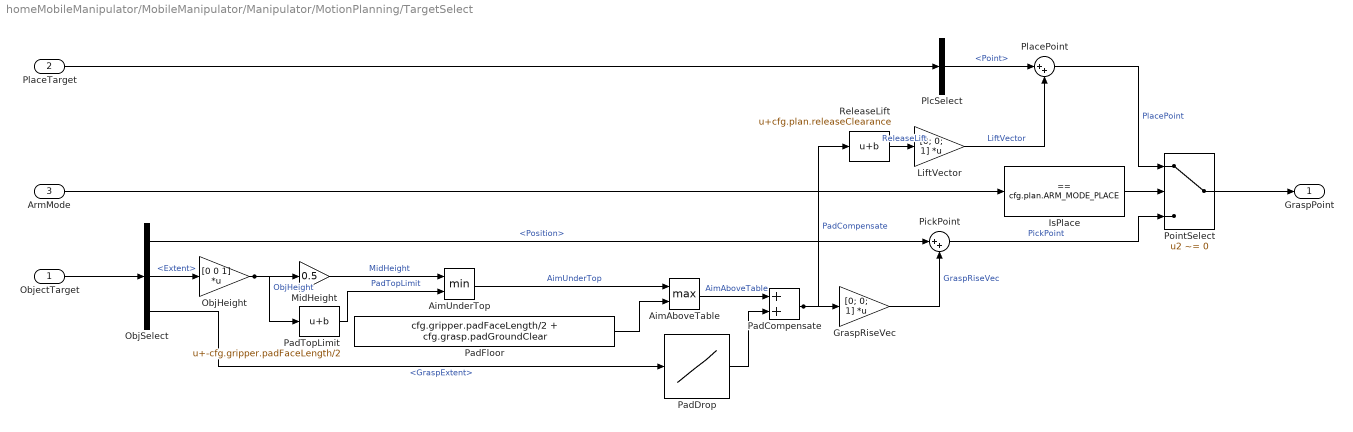
== system homeMobileManipulator/MobileManipulator/Manipulator/MotionPlanning/TargetSelect ==
  ObjectTarget : Inport  OutDataTypeStr=Bus: ObjectTarget
  PlaceTarget : Inport  Port=2  OutDataTypeStr=Bus: PlaceTarget
  ArmMode : Inport  Port=3  OutDataTypeStr=uint8
  AimAboveTable : MinMax  Description=max(AimUnderTop, PadFloor) -> the aim. THE FLOOR OUTRANKS THE CEILING, DELIBERATELY, and the max being outermost is what does it. The two can conflict on an object shorter than 2*(padFaceLength/2 + padGroundClear) = 57.5 mm, and they are not the same kind of fact: the support surface is real geometry the arm must not drive into, while the object top is a preference, and overshooting it only means part of the pad face stands clear while the rest still closes on the object. Above 57.5 mm this returns the mid-height exactly.  Function=max  Inputs=2
  AimUnderTop : MinMax  Description=min(MidHeight, PadTopLimit) - take the mid-height unless it would put the pad face over the object top.  Inputs=2
  GraspRiseVec : Gain  Gain=[0; 0; 1]  Multiplication=Matrix(K*u)
  IsPlace : hdlsllib/Logic and Bit Operations/Compare To Constant  relop===  const=cfg.plan.ARM_MODE_PLACE  OutDataTypeStr=boolean
  LiftVector : Gain  Gain=[0; 0; 1]  Multiplication=Matrix(K*u)
  MidHeight : Gain  Description=THE PREFERRED AIM: the jaws close across the MIDDLE of whatever they are given. Everything downstream of here is a bound on this number rather than a competing choice of it, which is why it is worth seeing on its own. A fixed fraction of the height (0.65) used to live here; a fraction scales the ground clearance with the object, so the clearance vanishes exactly when it matters.  Gain=0.5
  ObjHeight : Gain  Description=THE OBJECT HEIGHT, PULLED OUT OF THE EXTENT AS A SCALAR. [0 0 1] * Extent as a matrix product, so this is Extent(3) and nothing else. This block was GraspRise, a single Gain of [0 0 cfg.grasp.heightFraction] that turned the extent straight into the aim height. The aim is now a CLAMPED mid-height, so the bare height is needed first because two separate bounds are applied to it. The full reasoning is in hmmGraspAim, which is the one offline implementation of this same arithmetic.  Gain=[0 0 1]  Multiplication=Matrix(K*u)
  ObjSelect : BusSelector  OutputSignals=Position,Extent,GraspExtent
  PadCompensate : Sum  Description=THE TOOL RISE ABOVE THE SUPPORT SURFACE: the aim plus the pad drop. tcp_frame coincides with the pad-face centre only when the jaws are OPEN, so closing on an object drops the gripping surface below the tool frame by PadDrop(GraspExtent); adding it here is what makes the PAD land on the aim rather than the tool frame. ONE SUM FEEDS BOTH VERBS - GraspRiseVec for the pick and ReleaseLift for the place - and that sharing is the whole reason the release stays correct when the grasp height moves. It has moved three times and the place has never had to be re-derived.
  PadDrop : Lookup_n-D  Description=|  NumberOfTableDimensions=1  BreakpointsForDimension1=cfg.grasp.padDropWidth  Table=cfg.grasp.padDropTable  ExtrapMethod=Clip  InternalRulePriority=Speed  RndMeth=Simplest
      | Pad-face drop below tcp_frame, looked up on the object's jaw-axis width.
      | 
      | WHY THIS EXISTS. tcp_frame coincides with the pad-face centre only when the jaws are OPEN. Closing them swings the inner fingers and the pad face descends with the swing - 0.00 mm at the 92.4 mm open gap, 6.45 mm at the 74.4 mm gap the shipped mug closes to, 14.11 mm at a 19.3 mm gap, measured on armIkTree. Without this term the GRIPPING SURFACE lands up to 14 mm below the aim point, and always in the wrong direction: deeper, toward the table.
      | 
      | WHY A TABLE AND NOT A CONSTANT. The drop depends on how far the jaws close and that depends on the object, so a scalar would only be right for one object width. Breakpoints are jaw gaps; the driving signal is ObjectTarget.GraspExtent, the same width the capture gate matches on. Object width proxies the gap it closes to within about 1.2 mm on the shipped mug (jaws stop at 74.4 mm on a 70.0 mm object), and 1.2 mm against a 37.5 mm pad face does not justify a contact model.
      | 
      | Data: cfg.grasp.padDropWidth, cfg.grasp.padDropTable.
      | 
      | WHY THE ENDS CLAMP RATHER THAN EXTRAPOLATE. ExtrapMethod is Clip, not Linear. The table is
      | a MEASUREMENT over the aperture the pads were characterised at, so extending its end slope
      | would invent a contact geometry nobody measured - and off the TOP end it invents a NEGATIVE
      | pad drop, which moves the aim the wrong way: linear extrapolation to a 100 mm gap gives
      | -3.16 mm. This block shipped as Linear while the offline hmmGraspAim clamped, so the two were
      | not one rule. A gap sweep caught it only after it was made to leave the
      | breakpoints at both ends; INSIDE them every interpolation method agrees by construction, which
      | is why the first sweep reported no disagreement at all. Measured gap: 0.91 mm at a zero jaw
      | gap, 3.16 mm at 100 mm. No shipped prop reached it - the narrowest of the 20, PictureFrame, is
      | 21.0 mm against a 19.3 mm first breakpoint - but a narrower object is not impossible.
  PadFloor : Constant  Description=THE FLOOR: the lowest aim that keeps the pad face bottom edge cfg.grasp.padGroundClear = 10 mm above the support surface. Half the pad face, 18.75 mm, plus that clearance. A short object is not to be grasped by driving the jaws at the tabletop.  Value=cfg.gripper.padFaceLength/2 + cfg.grasp.padGroundClear
  PadTopLimit : Bias  Description=THE CEILING: the highest aim whose pad face still clears the object top. The pad face is cfg.gripper.padFaceLength = 37.5 mm tall, so it reaches half that above the aim point, and h - padFaceLength/2 is the aim at which its top edge touches the object top. NOTE FOR A READER: this term is provably INERT at every height for any non-negative cfg.grasp.padGroundClear, because below h = 2*padFaceLength/2 the floor downstream has already overridden it. It is kept because it is the written rule and both constraints the grasp respects should be visible here, but it is not doing work.  Bias=-cfg.gripper.padFaceLength/2  SaturateOnIntegerOverflow=off
  PickPoint : Sum  Inputs=|++
  PlacePoint : Sum  Inputs=|++
  PlcSelect : BusSelector  OutputSignals=Point
  PointSelect : Switch  Criteria=u2 ~= 0
  ReleaseLift : Bias  Bias=cfg.plan.releaseClearance
  GraspPoint : Outport
  wires:
  IsPlace/1 -> PointSelect/2
  PlacePoint/1 -> PointSelect/1  "PlacePoint"
  PointSelect/1 -> GraspPoint/1
  PickPoint/1 -> PointSelect/3  "PickPoint"
  LiftVector/1 -> PlacePoint/2  "LiftVector"
  GraspRiseVec/1 -> PickPoint/2  "GraspRiseVec"
  PlaceTarget/1 -> PlcSelect/1
  PadCompensate/1 -> GraspRiseVec/1, ReleaseLift/1  "PadCompensate"
  PadDrop/1 -> PadCompensate/2
  AimAboveTable/1 -> PadCompensate/1  "AimAboveTable"
  PlcSelect/1 -> PlacePoint/1  "<Point>"
  ObjHeight/1 -> MidHeight/1, PadTopLimit/1  "ObjHeight"
  AimUnderTop/1 -> AimAboveTable/1  "AimUnderTop"
  PadTopLimit/1 -> AimUnderTop/2  "PadTopLimit"
  ArmMode/1 -> IsPlace/1
  ObjSelect/2 -> ObjHeight/1  "<Extent>"
  MidHeight/1 -> AimUnderTop/1  "MidHeight"
  ReleaseLift/1 -> LiftVector/1  "ReleaseLift"
  ObjSelect/1 -> PickPoint/1  "<Position>"
  ObjectTarget/1 -> ObjSelect/1
  ObjSelect/3 -> PadDrop/1  "<GraspExtent>"
  PadFloor/1 -> AimAboveTable/2
